simulink model "sm_abbYuMi_trajectory"  (R2025a)
settings: Solver=daessc  StartTime=0.0  StopTime=size(waypointsL,2)*segment_duration  MaxStep=0.5  RelTol=1e-3  AbsTol=1e-3
values from neighbouring files (symbols this model uses):
  cube_l = 0.02    [startup_sm_abbYuMi_trajectory.m]
  segment_duration = 2    [startup_sm_abbYuMi_trajectory.m]
undefined symbols (not defined in the file or in its folder): F1, F2, X, Y, Z
libraries: sm_lib x210, nesl_utility x31, robotcorelib x2
(part 1 of 5)
CloseFcn:
  | try,close(h1_sm_abbYuMi_trajectory),end
  | clear h1_sm_abbYuMi_2_trajectory
  | try,close(h2_sm_abbYuMi_trajectory),end
  | clear h2_sm_abbYuMi_2_trajectory
  | try,close(h3_sm_abbYuMi_trajectory),end
  | clear h3_sm_abbYuMi_2_trajectory
  | try,close(h4_sm_abbYuMi_trajectory),end
  | clear h4_sm_abbYuMi_trajectory
  | 
  | 
  | clear simlog_sm_abbYuMi_trajectory
  | clear logsout_sm_abbYuMi_trajectory
Description:
  | Dual Arm Robot Trajectory Testing
  | Copyright 2021-2025 The MathWorks, Inc.
settings Model: Creator=smiller  LastModifiedBy=smiller
settings SolverCC: AutoScaleAbsTol=off
settings DataIOCC: MaxDataPoints=10000  ReturnWorkspaceOutputs=off  SignalLoggingName=logsout_sm_abbYuMi_trajectory
settings OptimizationCC: ReuseModelBlockBuffer=off
settings DebuggingCC: UnconnectedInputMsg=warning  UnconnectedOutputMsg=warning  UnconnectedLineMsg=warning
settings ModelReferenceCC: EnableRefExpFcnMdlSchedulingChecks=on
settings RTWCC: GPUComputeCapability=3.5  DLArmComputeVersion=19.05
settings SimscapeCC: SimscapeLogType=all  SimscapeLogSimulationStatistics=on  SimscapeLogName=simlog_sm_abbYuMi_trajectory  SimscapeLogDataHistory=10000.0
settings ExplorerConfigSet: InternalSimMechanicsExplorerSettings="<ExplorerConfiguration><canonicalview>default</canonicalview><AnimationSetting><BasePlaybackSpeed>1.0</BasePlaybackSpeed><PlaybackSpeedFactor>1.0</PlaybackSpeedFactor></AnimationSetting><TilePanel><TileInfo><Tiles Columns=\"3\" Count=\"4\" Rows=\"2\"><Column Weight=\"0.6174\"/><Column Weight=\"0.1908\"/><Column Weight=\"0.1918\"/><Row Weight=\"0.4992\"/><Row Weight=\"0.5008\"/><Tile Height=\"2\" Width=\"1\" X=\"0\" Y=\"0\"/><Tile Height=\"1\" Width=\"1\" X=\"1\" Y=\"0\"/><Tile Height=\"1\" Width=\"1\" X=\"2\" Y=\"0\"/><Tile Height=\"1\" Width=\"2\" X=\"1\" Y=\"1\"/></Tiles></TileInfo><SceneInfo><SceneViewer><BGColor><R>1</R><G>1</G><B>1</B></BGColor><Camera><DoPerspective>off</DoPerspective><Position><X>1.10785151491655953</X><Y>0.401938303575801459</Y><Z>0.73930542035196356</Z></Position><Center><X>0.0422085680859981827</X><Y>-0.0186832884618209454</Y><Z>0.276020887594053299</Z></Center><Up><X>-0.346127033108781346</X><Y>-0.144162748431228449</Y><Z>0.927045402834222987</Z></Up><ViewLimDist>1</ViewLimDist><YLim>0.529480286240577747</YLim><XLim>0.750259888990338908</XLim></Camera></SceneViewer><SceneViewer><BGColor><R>1</R><G>1</G><B>1</B></BGColor><Camera><DoPerspective>off</DoPerspective><Position><X>1.28857080950961111</X><Y>0.165761602408297848</Y><Z>0.538044175913367062</Z></Position><Center><X>0.222927862679049932</X><Y>-0.254859989629324657</Y><Z>0.0747596431554567176</Z></Center><Up><X>-0.346127033108781346</X><Y>-0.144162748431228449</Y><Z>0.927045402834222987</Z></Up><ViewLimDist>1</ViewLimDist><YLim>0.0401775125475980072</YLim><XLim>0.0353441275794659157</XLim></Camera></SceneViewer><SceneViewer><BGColor><R>1</R><G>1</G><B>1</B></BGColor><Camera><DoPerspective>off</DoPerspective><Position><X>1.11107526675001367</X><Y>0.699993298566071065</Y><Z>0.461282465118678986</Z></Position><Center><X>0.045432319919452957</X><Y>0.279371706528448394</Y><Z>-0.002002067639231578</Z></Center><Up><X>-0.346127033108781346</X><Y>-0.144162748431228449</Y><Z>0.927045402834222987</Z></Up><ViewLimDist>1</ViewLimDist><YLim>0.0406072638280753281</YLim><XLim>0.0358748383443522681</XLim></Camera></SceneViewer><SceneViewer><BGColor><R>1</R><G>1</G><B>1</B></BGColor><Camera><DoPerspective>off</DoPerspective><Position><X>1.27319716760923374</X><Y>0.344894477488872697</Y><Z>0.410769600840851012</Z></Position><Center><X>0.207554220778672804</X><Y>-0.0757271145487498354</Y><Z>-0.0525149319170593112</Z></Center><Up><X>-0.346127033108781346</X><Y>-0.144162748431228449</Y><Z>0.927045402834222987</Z></Up><ViewLimDist>1</ViewLimDist><YLim>0.0389773841730341117</YLim><XLim>0.0697797364595891534</XLim></Camera></SceneViewer></SceneInfo></TilePanel><MechEditorPanel><Cameras/><GfxPanelCameraMap/><VideoCreator><PlaybackSpeedRatio>1</PlaybackSpeedRatio><FrameRate>30</FrameRate><VideoFormat>MPEG-4</VideoFormat><FrameSize>auto</FrameSize></VideoCreator></MechEditorPanel></ExplorerConfiguration>"

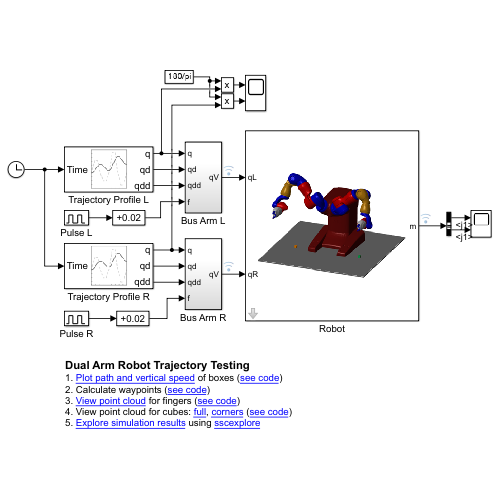
[thumbnail: Simulink's stored preview of the top-level diagram]
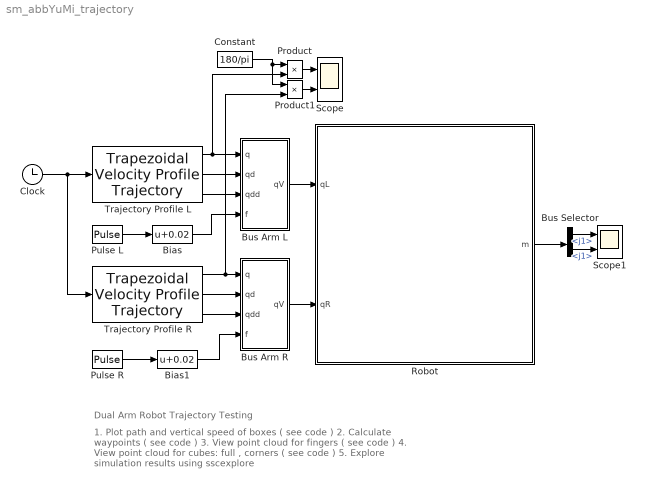
== system sm_abbYuMi_trajectory ==
  note: Dual Arm Robot Trajectory Testing
  note: 1. Plot path and vertical speed of boxes ( see code )
      | 2. Calculate waypoints ( see code )
      | 3. View point cloud for fingers ( see code )
      | 4. View point cloud for cubes: full , corners ( see code )
      | 5. Explore simulation results using sscexplore
  Bias : Bias  Bias=0.02  SaturateOnIntegerOverflow=off
  Bias1 : Bias  Bias=0.02  SaturateOnIntegerOverflow=off
  Bus Selector : BusSelector  OutputSignals=trqL.j1,trqR.j1
  Bus Arm L : Subsystem
  Bus Arm R : Subsystem
  Clock : Clock
  Constant : Constant  Value=180/pi
  Product : Product
  Product1 : Product
  Pulse L : DiscretePulseGenerator  PulseType=Time based  Amplitude=-0.011  Period=100  PulseWidth=4*segment_duration  PhaseDelay=2*segment_duration
  Pulse R : DiscretePulseGenerator  PulseType=Time based  Amplitude=-0.011  Period=100  PulseWidth=4*segment_duration  PhaseDelay=6*segment_duration
  Robot : Subsystem  mask(Dual Arm Robot with Contact Forces){k_gripBox=1e3, k_boxBox=1e3, k_boxFloor=1e3, d_gripBox=1e2, d_boxBox=1e2, d_boxFloor=1e2, t_gripBox=1e-3, t_boxBox=1e-3, t_boxFloor=1e-3, mu_s_gripBox=0.7, mu_s_boxBox=0.5, mu_s_boxFloor=0.5, mu_d_gripBox=0.5, mu_d_boxBox=0.3, mu_d_boxFloor=0.3, mu_v_gripBox=1e-3, mu_v_boxBox=1e-3, mu_v_boxFloor=1e-3}
      mask help: Models a dual-arm robot. Parameter values define the contact and friction forces between the gripper, boxes, and floor.
      mask DialogControl Control2_copy_copy_copy_copy_copy_copy_copy Prompt: Gripper-Box
      mask DialogControl Control2_copy_copy_copy_copy_copy_copy_copy_copy Prompt: Box-Box
      mask DialogControl Control2_copy_copy_copy_copy_copy_copy_copy_copy_copy Prompt: Box-Floor
      mask DialogControl Control2_copy_copy_copy_copy_copy_copy Prompt: Damping (N/(m/s))
      mask DialogControl Control2_copy Prompt: Damping (N/(m/s))
      mask DialogControl Control2_copy_copy Prompt: Transition Width (m)
      mask DialogControl Control2_copy_copy_copy Prompt: Static Friction (0-1)
      mask DialogControl Control2_copy_copy_copy_copy Prompt: Dynamic Friction (0-1)
      mask DialogControl Control2_copy_copy_copy_copy_copy Prompt: Critical Velocity (m/s)
      mask Display: image('sm_abbYuMi_trajectory_robot.png');
  Scope : Scope  NumInputPorts=2
      settings: ActiveDisplayYMinimum=-224.28794  ActiveDisplayYMaximum=180.85767
  Scope1 : Scope  NumInputPorts=2
      settings: ActiveDisplayYMinimum=-24.11191  ActiveDisplayYMaximum=24.30925
  Trajectory Profile L : robotcorelib/Trapezoidal Velocity Profile Trajectory  WaypointSource=Internal  Waypoints=waypointsL  NumParams=1  Parameter1=End Time  Parameter2=End Time  ParameterSource=Internal  PeakVelocity=[ 2; 2 ]  Acceleration=[ 1; 2 ]  EndTime=segment_duration  AccelTime=[ 1; 2 ]  SimulateUsing=Code generation
  Trajectory Profile R : robotcorelib/Trapezoidal Velocity Profile Trajectory  WaypointSource=Internal  Waypoints=waypointsR  NumParams=1  Parameter1=End Time  Parameter2=End Time  ParameterSource=Internal  PeakVelocity=[ 2; 2 ]  Acceleration=[ 1; 2 ]  EndTime=segment_duration  AccelTime=[ 1; 2 ]  SimulateUsing=Code generation
  wires:
  Clock/1 -> Trajectory Profile R/1, Trajectory Profile L/1
  Trajectory Profile L/1 -> Product/2, Bus Arm L/1(q)
  Trajectory Profile L/2 -> Bus Arm L/2(qd)
  Trajectory Profile L/3 -> Bus Arm L/3(qdd)
  Product/1 -> Scope/1
  Pulse L/1 -> Bias/1
  Trajectory Profile R/3 -> Bus Arm R/3(qdd)
  Trajectory Profile R/2 -> Bus Arm R/2(qd)
  Trajectory Profile R/1 -> Product1/2, Bus Arm R/1(q)
  Product1/1 -> Scope/2
  Pulse R/1 -> Bias1/1
  Bus Arm L/1(qV) -> Robot/1(qL)
  Bus Arm R/1(qV) -> Robot/2(qR)
  Constant/1 -> Product1/1, Product/1
  Bias1/1 -> Bus Arm R/4(f)
  Bias/1 -> Bus Arm L/4(f)
  Robot/1(m) -> Bus Selector/1
  Bus Selector/1 -> Scope1/1  "<j1>"
  Bus Selector/2 -> Scope1/2  "<j1>"

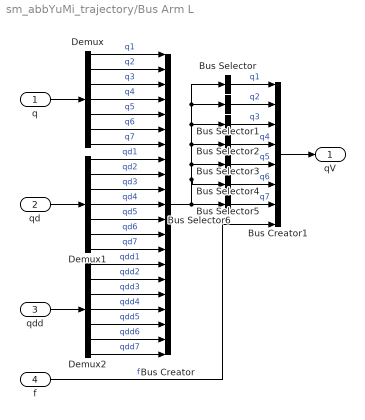
== system sm_abbYuMi_trajectory/Bus Arm L ==
  q : Inport
  qd : Inport  Port=2
  qdd : Inport  Port=3
  f : Inport  Port=4
  Bus Creator : BusCreator  Inputs=21
  Bus Creator1 : BusCreator  Inputs=8
  Bus Selector : BusSelector  OutputSignals=q1,qd1,qdd1  OutputAsBus=on
  Bus Selector1 : BusSelector  OutputSignals=q2,qd2,qdd2  OutputAsBus=on
  Bus Selector2 : BusSelector  OutputSignals=q3,qd3,qdd3  OutputAsBus=on
  Bus Selector3 : BusSelector  OutputSignals=q4,qd4,qdd4  OutputAsBus=on
  Bus Selector4 : BusSelector  OutputSignals=q5,qd5,qdd5  OutputAsBus=on
  Bus Selector5 : BusSelector  OutputSignals=q6,qd6,qdd6  OutputAsBus=on
  Bus Selector6 : BusSelector  OutputSignals=q7,qd7,qdd7  OutputAsBus=on
  Demux : Demux  Outputs=7
  Demux1 : Demux  Outputs=7
  Demux2 : Demux  Outputs=7
  qV : Outport
  wires:
  f/1 -> Bus Creator1/8  "f"
  q/1 -> Demux/1
  qd/1 -> Demux1/1
  qdd/1 -> Demux2/1
  Demux/1 -> Bus Creator/1  "q1"
  Demux/2 -> Bus Creator/2  "q2"
  Demux/3 -> Bus Creator/3  "q3"
  Demux/4 -> Bus Creator/4  "q4"
  Demux/5 -> Bus Creator/5  "q5"
  Demux/6 -> Bus Creator/6  "q6"
  Demux/7 -> Bus Creator/7  "q7"
  Demux1/1 -> Bus Creator/8  "qd1"
  Demux1/2 -> Bus Creator/9  "qd2"
  Demux1/3 -> Bus Creator/10  "qd3"
  Demux1/4 -> Bus Creator/11  "qd4"
  Demux1/5 -> Bus Creator/12  "qd5"
  Demux1/6 -> Bus Creator/13  "qd6"
  Demux1/7 -> Bus Creator/14  "qd7"
  Demux2/1 -> Bus Creator/15  "qdd1"
  Demux2/2 -> Bus Creator/16  "qdd2"
  Demux2/3 -> Bus Creator/17  "qdd3"
  Demux2/4 -> Bus Creator/18  "qdd4"
  Demux2/5 -> Bus Creator/19  "qdd5"
  Demux2/6 -> Bus Creator/20  "qdd6"
  Demux2/7 -> Bus Creator/21  "qdd7"
  Bus Creator/1 -> Bus Selector5/1, Bus Selector4/1, Bus Selector3/1, Bus Selector2/1, Bus Selector/1, Bus Selector1/1, Bus Selector6/1
  Bus Selector/1 -> Bus Creator1/1  "q1"
  Bus Selector1/1 -> Bus Creator1/2  "q2"
  Bus Selector2/1 -> Bus Creator1/3  "q3"
  Bus Selector3/1 -> Bus Creator1/4  "q4"
  Bus Selector4/1 -> Bus Creator1/5  "q5"
  Bus Selector5/1 -> Bus Creator1/6  "q6"
  Bus Selector6/1 -> Bus Creator1/7  "q7"
  Bus Creator1/1 -> qV/1

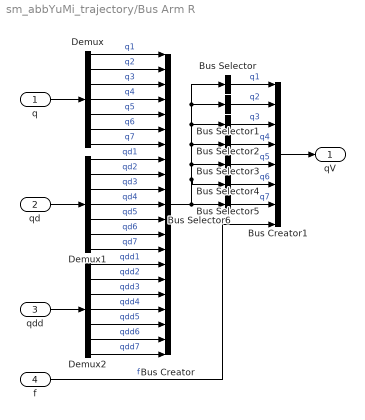
== system sm_abbYuMi_trajectory/Bus Arm R ==
  q : Inport
  qd : Inport  Port=2
  qdd : Inport  Port=3
  f : Inport  Port=4
  Bus Creator : BusCreator  Inputs=21
  Bus Creator1 : BusCreator  Inputs=8
  Bus Selector : BusSelector  OutputSignals=q1,qd1,qdd1  OutputAsBus=on
  Bus Selector1 : BusSelector  OutputSignals=q2,qd2,qdd2  OutputAsBus=on
  Bus Selector2 : BusSelector  OutputSignals=q3,qd3,qdd3  OutputAsBus=on
  Bus Selector3 : BusSelector  OutputSignals=q4,qd4,qdd4  OutputAsBus=on
  Bus Selector4 : BusSelector  OutputSignals=q5,qd5,qdd5  OutputAsBus=on
  Bus Selector5 : BusSelector  OutputSignals=q6,qd6,qdd6  OutputAsBus=on
  Bus Selector6 : BusSelector  OutputSignals=q7,qd7,qdd7  OutputAsBus=on
  Demux : Demux  Outputs=7
  Demux1 : Demux  Outputs=7
  Demux2 : Demux  Outputs=7
  qV : Outport
  wires:
  Bus Creator1/1 -> qV/1
  Bus Selector6/1 -> Bus Creator1/7  "q7"
  Bus Selector5/1 -> Bus Creator1/6  "q6"
  Bus Selector4/1 -> Bus Creator1/5  "q5"
  Bus Selector3/1 -> Bus Creator1/4  "q4"
  Bus Selector2/1 -> Bus Creator1/3  "q3"
  Bus Selector1/1 -> Bus Creator1/2  "q2"
  Bus Selector/1 -> Bus Creator1/1  "q1"
  Bus Creator/1 -> Bus Selector6/1, Bus Selector1/1, Bus Selector/1, Bus Selector2/1, Bus Selector3/1, Bus Selector4/1, Bus Selector5/1
  Demux2/7 -> Bus Creator/21  "qdd7"
  Demux2/6 -> Bus Creator/20  "qdd6"
  Demux2/5 -> Bus Creator/19  "qdd5"
  Demux2/4 -> Bus Creator/18  "qdd4"
  Demux2/3 -> Bus Creator/17  "qdd3"
  Demux2/2 -> Bus Creator/16  "qdd2"
  Demux2/1 -> Bus Creator/15  "qdd1"
  Demux1/7 -> Bus Creator/14  "qd7"
  Demux1/6 -> Bus Creator/13  "qd6"
  Demux1/5 -> Bus Creator/12  "qd5"
  Demux1/4 -> Bus Creator/11  "qd4"
  Demux1/3 -> Bus Creator/10  "qd3"
  Demux1/2 -> Bus Creator/9  "qd2"
  Demux1/1 -> Bus Creator/8  "qd1"
  Demux/7 -> Bus Creator/7  "q7"
  Demux/6 -> Bus Creator/6  "q6"
  Demux/5 -> Bus Creator/5  "q5"
  Demux/4 -> Bus Creator/4  "q4"
  Demux/3 -> Bus Creator/3  "q3"
  Demux/2 -> Bus Creator/2  "q2"
  Demux/1 -> Bus Creator/1  "q1"
  qdd/1 -> Demux2/1
  qd/1 -> Demux1/1
  q/1 -> Demux/1
  f/1 -> Bus Creator1/8  "f"

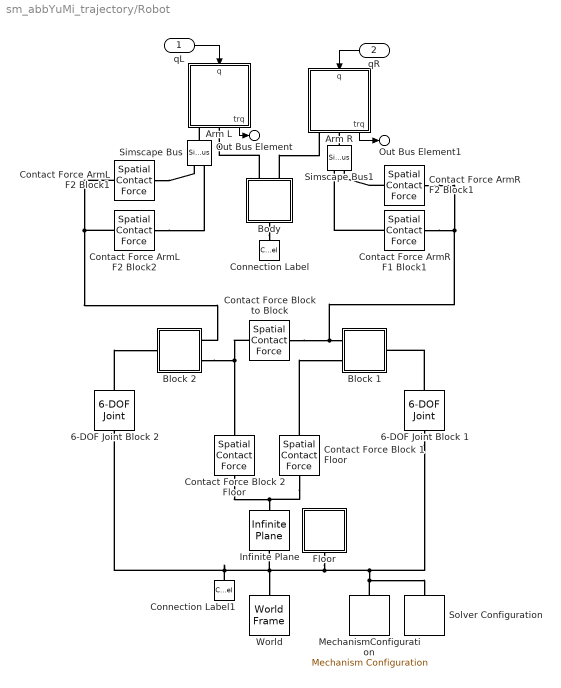
== system sm_abbYuMi_trajectory/Robot ==
  qL : Inport
  qR : Inport  Port=2
  " Contact Force Block to Block" : sm_lib/Forces and Torques/Spatial Contact Force  SenseSeparationDistance=off  NormalForceType=SmoothSpringDamper  NormalStiffness=k_boxBox  NormalStiffnessUnits=N/m  NormalDamping=d_boxBox  NormalDampingUnits=N/(m/s)  NormalTransitionRegionWidth=t_boxBox  NormalTransitionRegionWidthUnits=m  FrictionType=SmoothStickSlip  CoefficientOfStaticFriction=mu_s_boxBox  CoefficientOfDynamicFriction=mu_d_boxBox  FrictionalCriticalVelocity=mu_v_boxBox  FrictionalCriticalVelocityUnits=m/s  SenseContactSignal=off  SensePenetrationDepth=off  SenseNormalVelocity=off  SenseTangentialVelocity=off  SensingForceTorqueDirection=BaseOnFollower  SensingForceTorqueResolutionFrame=ContactFrame  SenseNormalForce=off  SenseNormalForceMagnitude=off  SenseNormalTorque=off  SenseFrictionalForce=off  SenseFrictionalForceMagnitude=off  SenseFrictionalTorque=off  SenseTotalForce=off  SenseTotalTorque=off  SenseContactBaseRotation=off  SenseContactBaseTranslation=off  SenseContactFollowerRotation=off  SenseContactFollowerTranslation=off  ZeroCrossDetectContactStartAndEnd=off
  6-DOF Joint Block 1 : sm_lib/Joints/6-DOF Joint  JointMode=Normal  CompositeWrenchDir=FollowerOnBase  CompositeWrenchFrame=BaseFrame  SenseConstraintForce=off  SenseConstraintTorque=off  SenseTotalForce=off  SenseTotalTorque=off  PxPositionTargetSpecify=on  PxPositionTargetPriority=High  PxPositionTargetValue=0.1  PxPositionTargetValueUnits=m  PxVelocityTargetSpecify=off  PxVelocityTargetPriority=High  PxVelocityTargetValue=0  PxVelocityTargetValueUnits=m/s  PxEquilibriumPosition=0  PxEquilibriumPositionUnits=m  PxSpringStiffness=0  PxSpringStiffnessUnits=N/m  PxDampingCoefficient=0  PxDampingCoefficientUnits=N/(m/s)  PxLowerLimitSpecify=off  PxLowerLimitBound=-1  PxLowerLimitBoundUnits=m  PxLowerLimitStiffness=1e6  PxLowerLimitStiffnessUnits=N/m  PxLowerLimitDamping=1e3  PxLowerLimitDampingUnits=N/(m/s)  PxLowerLimitTransitionRegionWidth=1e-4  PxLowerLimitTransitionRegionWidthUnits=m  PxUpperLimitSpecify=off  PxUpperLimitBound=1  PxUpperLimitBoundUnits=m  PxUpperLimitStiffness=1e6  PxUpperLimitStiffnessUnits=N/m  PxUpperLimitDamping=1e3  PxUpperLimitDampingUnits=N/(m/s)  PxUpperLimitTransitionRegionWidth=1e-4  PxUpperLimitTransitionRegionWidthUnits=m  PxTorqueActuationMode=NoTorque  PxMotionActuationMode=ComputedMotion  PxSensePosition=off  PxSenseVelocity=off  PxSenseAcceleration=off  PxSenseTorqueForce=off  PxSenseLowerLimitTorqueForce=off  PxSenseUpperLimitTorqueForce=off  PyPositionTargetSpecify=on  PyPositionTargetPriority=High  PyPositionTargetValue=-0.3  PyPositionTargetValueUnits=m  PyVelocityTargetSpecify=off  PyVelocityTargetPriority=High  PyVelocityTargetValue=0  PyVelocityTargetValueUnits=m/s  PyEquilibriumPosition=0  PyEquilibriumPositionUnits=m  PySpringStiffness=0  PySpringStiffnessUnits=N/m  PyDampingCoefficient=0  PyDampingCoefficientUnits=N/(m/s)  PyLowerLimitSpecify=off  PyLowerLimitBound=-1  PyLowerLimitBoundUnits=m  PyLowerLimitStiffness=1e6  PyLowerLimitStiffnessUnits=N/m  PyLowerLimitDamping=1e3  PyLowerLimitDampingUnits=N/(m/s)  PyLowerLimitTransitionRegionWidth=1e-4  PyLowerLimitTransitionRegionWidthUnits=m  PyUpperLimitSpecify=off  PyUpperLimitBound=1  PyUpperLimitBoundUnits=m  PyUpperLimitStiffness=1e6  PyUpperLimitStiffnessUnits=N/m  PyUpperLimitDamping=1e3  PyUpperLimitDampingUnits=N/(m/s)  PyUpperLimitTransitionRegionWidth=1e-4  PyUpperLimitTransitionRegionWidthUnits=m  PyTorqueActuationMode=NoTorque  PyMotionActuationMode=ComputedMotion  PySensePosition=off  PySenseVelocity=off  PySenseAcceleration=off  PySenseTorqueForce=off  PySenseLowerLimitTorqueForce=off  PySenseUpperLimitTorqueForce=off  PzPositionTargetSpecify=on  PzPositionTargetPriority=High  PzPositionTargetValue=0.011  PzPositionTargetValueUnits=m  PzVelocityTargetSpecify=off  PzVelocityTargetPriority=High  PzVelocityTargetValue=0  PzVelocityTargetValueUnits=m/s  PzEquilibriumPosition=0  PzEquilibriumPositionUnits=m  PzSpringStiffness=0  PzSpringStiffnessUnits=N/m  PzDampingCoefficient=0  PzDampingCoefficientUnits=N/(m/s)  PzLowerLimitSpecify=off  PzLowerLimitBound=0  PzLowerLimitBoundUnits=m  PzLowerLimitStiffness=1e6  PzLowerLimitStiffnessUnits=N/m  PzLowerLimitDamping=1e3  PzLowerLimitDampingUnits=N/(m/s)  PzLowerLimitTransitionRegionWidth=1e-4  PzLowerLimitTransitionRegionWidthUnits=m  PzUpperLimitSpecify=off  PzUpperLimitBound=1  PzUpperLimitBoundUnits=m  PzUpperLimitStiffness=1e6  PzUpperLimitStiffnessUnits=N/m  PzUpperLimitDamping=1e3  PzUpperLimitDampingUnits=N/(m/s)  PzUpperLimitTransitionRegionWidth=1e-4  PzUpperLimitTransitionRegionWidthUnits=m  PzTorqueActuationMode=NoTorque  PzMotionActuationMode=ComputedMotion  PzSensePosition=off  PzSenseVelocity=off  PzSenseAcceleration=off  PzSenseTorqueForce=off  PzSenseLowerLimitTorqueForce=off  PzSenseUpperLimitTorqueForce=off  SphPositionTargetSpecify=off  SphPositionTargetPriority=High  SphPositionTargetRotationMethod=None  SphPositionTargetFollAlignAxisA=+X  SphPositionTargetBaseAlignAxisA=+Y  SphPositionTargetFollAlignAxisB=+Y  SphPositionTargetBaseAlignAxisB=+Z  SphPositionTargetRotationStandardAxis=+Z  SphPositionTargetRotationAngle=0.0  SphPositionTargetRotationAngleUnits=deg  SphPositionTargetRotationArbitraryAxis=[0 0 1]  SphPositionTargetRotationSequenceAxes=FollowerAxes  SphPositionTargetRotationSequence=XYX  SphPositionTargetRotationSequenceAngles=[0 0 0]  SphPositionTargetRotationSequenceAnglesUnits=deg  SphPositionTargetRotationMatrix=[1 0 0; 0 1 0; 0 0 1]  SphPositionTargetQuaternion=[1 0 0 0]  SphVelocityTargetSpecify=off  SphVelocityTargetPriority=High  SphVelocityTargetValue=[0 0 0]  SphVelocityTargetValueUnits=deg/s  SphVelocityTargetInFollowerFrame=on  SphEqPosRotationMethod=None  SphEqPosFollAlignAxisA=+X  SphEqPosBaseAlignAxisA=+Y  SphEqPosFollAlignAxisB=+Y  SphEqPosBaseAlignAxisB=+Z  SphEqPosRotationStandardAxis=+Z  SphEqPosRotationAngle=0.0  SphEqPosRotationAngleUnits=deg  SphEqPosRotationArbitraryAxis=[0 0 1]  SphEqPosRotationSequenceAxes=FollowerAxes  SphEqPosRotationSequence=XYX  SphEqPosRotationSequenceAngles=[0 0 0]  SphEqPosRotationSequenceAnglesUnits=deg  SphEqPosRotationMatrix=[1 0 0; 0 1 0; 0 0 1]  SphEqPosQuaternion=[1 0 0 0]  SphSpringStiffness=0  SphSpringStiffnessUnits=N*m/deg  SphDampingCoefficient=0  SphDampingCoefficientUnits=N*m/(deg/s)  SphLowerLimitSpecify=off  SphLowerLimitBound=15  SphLowerLimitBoundUnits=deg  SphLowerLimitStiffness=1e4  SphLowerLimitStiffnessUnits=N*m/deg  SphLowerLimitDamping=10  SphLowerLimitDampingUnits=N*m/(deg/s)  SphLowerLimitTransitionRegionWidth=0.1  SphLowerLimitTransitionRegionWidthUnits=deg  SphUpperLimitSpecify=off  SphUpperLimitBound=45  SphUpperLimitBoundUnits=deg  SphUpperLimitStiffness=1e4  SphUpperLimitStiffnessUnits=N*m/deg  SphUpperLimitDamping=10  SphUpperLimitDampingUnits=N*m/(deg/s)  SphUpperLimitTransitionRegionWidth=0.1  SphUpperLimitTransitionRegionWidthUnits=deg  SphTorqueActuationMode=NoTorque  SphActuateTorqueX=off  SphActuateTorqueY=off  SphActuateTorqueZ=off  SphActuateTorque=off  SphActuationFrame=BaseFrame  SphSensePosition=off  SphSenseVelocityX=off  SphSenseVelocityY=off  SphSenseVelocityZ=off  SphSenseVelocity=off  SphSenseAccelerationX=off  SphSenseAccelerationY=off  SphSenseAccelerationZ=off  SphSenseAcceleration=off  SphSenseLowerLimitTorqueMag=off  SphSenseUpperLimitTorqueMag=off  SphSensingFrame=BaseFrame
  6-DOF Joint Block 2 : sm_lib/Joints/6-DOF Joint  JointMode=Normal  CompositeWrenchDir=FollowerOnBase  CompositeWrenchFrame=BaseFrame  SenseConstraintForce=off  SenseConstraintTorque=off  SenseTotalForce=off  SenseTotalTorque=off  PxPositionTargetSpecify=on  PxPositionTargetPriority=High  PxPositionTargetValue=0.1  PxPositionTargetValueUnits=m  PxVelocityTargetSpecify=off  PxVelocityTargetPriority=High  PxVelocityTargetValue=0  PxVelocityTargetValueUnits=m/s  PxEquilibriumPosition=0  PxEquilibriumPositionUnits=m  PxSpringStiffness=0  PxSpringStiffnessUnits=N/m  PxDampingCoefficient=0  PxDampingCoefficientUnits=N/(m/s)  PxLowerLimitSpecify=off  PxLowerLimitBound=-1  PxLowerLimitBoundUnits=m  PxLowerLimitStiffness=1e6  PxLowerLimitStiffnessUnits=N/m  PxLowerLimitDamping=1e3  PxLowerLimitDampingUnits=N/(m/s)  PxLowerLimitTransitionRegionWidth=1e-4  PxLowerLimitTransitionRegionWidthUnits=m  PxUpperLimitSpecify=off  PxUpperLimitBound=1  PxUpperLimitBoundUnits=m  PxUpperLimitStiffness=1e6  PxUpperLimitStiffnessUnits=N/m  PxUpperLimitDamping=1e3  PxUpperLimitDampingUnits=N/(m/s)  PxUpperLimitTransitionRegionWidth=1e-4  PxUpperLimitTransitionRegionWidthUnits=m  PxTorqueActuationMode=NoTorque  PxMotionActuationMode=ComputedMotion  PxSensePosition=off  PxSenseVelocity=off  PxSenseAcceleration=off  PxSenseTorqueForce=off  PxSenseLowerLimitTorqueForce=off  PxSenseUpperLimitTorqueForce=off  PyPositionTargetSpecify=on  PyPositionTargetPriority=High  PyPositionTargetValue=0.3  PyPositionTargetValueUnits=m  PyVelocityTargetSpecify=off  PyVelocityTargetPriority=High  PyVelocityTargetValue=0  PyVelocityTargetValueUnits=m/s  PyEquilibriumPosition=0  PyEquilibriumPositionUnits=m  PySpringStiffness=0  PySpringStiffnessUnits=N/m  PyDampingCoefficient=0  PyDampingCoefficientUnits=N/(m/s)  PyLowerLimitSpecify=off  PyLowerLimitBound=-1  PyLowerLimitBoundUnits=m  PyLowerLimitStiffness=1e6  PyLowerLimitStiffnessUnits=N/m  PyLowerLimitDamping=1e3  PyLowerLimitDampingUnits=N/(m/s)  PyLowerLimitTransitionRegionWidth=1e-4  PyLowerLimitTransitionRegionWidthUnits=m  PyUpperLimitSpecify=off  PyUpperLimitBound=1  PyUpperLimitBoundUnits=m  PyUpperLimitStiffness=1e6  PyUpperLimitStiffnessUnits=N/m  PyUpperLimitDamping=1e3  PyUpperLimitDampingUnits=N/(m/s)  PyUpperLimitTransitionRegionWidth=1e-4  PyUpperLimitTransitionRegionWidthUnits=m  PyTorqueActuationMode=NoTorque  PyMotionActuationMode=ComputedMotion  PySensePosition=off  PySenseVelocity=off  PySenseAcceleration=off  PySenseTorqueForce=off  PySenseLowerLimitTorqueForce=off  PySenseUpperLimitTorqueForce=off  PzPositionTargetSpecify=on  PzPositionTargetPriority=High  PzPositionTargetValue=0.011  PzPositionTargetValueUnits=m  PzVelocityTargetSpecify=off  PzVelocityTargetPriority=High  PzVelocityTargetValue=0  PzVelocityTargetValueUnits=m/s  PzEquilibriumPosition=0  PzEquilibriumPositionUnits=m  PzSpringStiffness=0  PzSpringStiffnessUnits=N/m  PzDampingCoefficient=0  PzDampingCoefficientUnits=N/(m/s)  PzLowerLimitSpecify=off  PzLowerLimitBound=0  PzLowerLimitBoundUnits=m  PzLowerLimitStiffness=1e6  PzLowerLimitStiffnessUnits=N/m  PzLowerLimitDamping=1e3  PzLowerLimitDampingUnits=N/(m/s)  PzLowerLimitTransitionRegionWidth=1e-4  PzLowerLimitTransitionRegionWidthUnits=m  PzUpperLimitSpecify=off  PzUpperLimitBound=1  PzUpperLimitBoundUnits=m  PzUpperLimitStiffness=1e6  PzUpperLimitStiffnessUnits=N/m  PzUpperLimitDamping=1e3  PzUpperLimitDampingUnits=N/(m/s)  PzUpperLimitTransitionRegionWidth=1e-4  PzUpperLimitTransitionRegionWidthUnits=m  PzTorqueActuationMode=NoTorque  PzMotionActuationMode=ComputedMotion  PzSensePosition=off  PzSenseVelocity=off  PzSenseAcceleration=off  PzSenseTorqueForce=off  PzSenseLowerLimitTorqueForce=off  PzSenseUpperLimitTorqueForce=off  SphPositionTargetSpecify=off  SphPositionTargetPriority=High  SphPositionTargetRotationMethod=None  SphPositionTargetFollAlignAxisA=+X  SphPositionTargetBaseAlignAxisA=+Y  SphPositionTargetFollAlignAxisB=+Y  SphPositionTargetBaseAlignAxisB=+Z  SphPositionTargetRotationStandardAxis=+Z  SphPositionTargetRotationAngle=0.0  SphPositionTargetRotationAngleUnits=deg  SphPositionTargetRotationArbitraryAxis=[0 0 1]  SphPositionTargetRotationSequenceAxes=FollowerAxes  SphPositionTargetRotationSequence=XYX  SphPositionTargetRotationSequenceAngles=[0 0 0]  SphPositionTargetRotationSequenceAnglesUnits=deg  SphPositionTargetRotationMatrix=[1 0 0; 0 1 0; 0 0 1]  SphPositionTargetQuaternion=[1 0 0 0]  SphVelocityTargetSpecify=off  SphVelocityTargetPriority=High  SphVelocityTargetValue=[0 0 0]  SphVelocityTargetValueUnits=deg/s  SphVelocityTargetInFollowerFrame=on  SphEqPosRotationMethod=None  SphEqPosFollAlignAxisA=+X  SphEqPosBaseAlignAxisA=+Y  SphEqPosFollAlignAxisB=+Y  SphEqPosBaseAlignAxisB=+Z  SphEqPosRotationStandardAxis=+Z  SphEqPosRotationAngle=0.0  SphEqPosRotationAngleUnits=deg  SphEqPosRotationArbitraryAxis=[0 0 1]  SphEqPosRotationSequenceAxes=FollowerAxes  SphEqPosRotationSequence=XYX  SphEqPosRotationSequenceAngles=[0 0 0]  SphEqPosRotationSequenceAnglesUnits=deg  SphEqPosRotationMatrix=[1 0 0; 0 1 0; 0 0 1]  SphEqPosQuaternion=[1 0 0 0]  SphSpringStiffness=0  SphSpringStiffnessUnits=N*m/deg  SphDampingCoefficient=0  SphDampingCoefficientUnits=N*m/(deg/s)  SphLowerLimitSpecify=off  SphLowerLimitBound=15  SphLowerLimitBoundUnits=deg  SphLowerLimitStiffness=1e4  SphLowerLimitStiffnessUnits=N*m/deg  SphLowerLimitDamping=10  SphLowerLimitDampingUnits=N*m/(deg/s)  SphLowerLimitTransitionRegionWidth=0.1  SphLowerLimitTransitionRegionWidthUnits=deg  SphUpperLimitSpecify=off  SphUpperLimitBound=45  SphUpperLimitBoundUnits=deg  SphUpperLimitStiffness=1e4  SphUpperLimitStiffnessUnits=N*m/deg  SphUpperLimitDamping=10  SphUpperLimitDampingUnits=N*m/(deg/s)  SphUpperLimitTransitionRegionWidth=0.1  SphUpperLimitTransitionRegionWidthUnits=deg  SphTorqueActuationMode=NoTorque  SphActuateTorqueX=off  SphActuateTorqueY=off  SphActuateTorqueZ=off  SphActuateTorque=off  SphActuationFrame=BaseFrame  SphSensePosition=off  SphSenseVelocityX=off  SphSenseVelocityY=off  SphSenseVelocityZ=off  SphSenseVelocity=off  SphSenseAccelerationX=off  SphSenseAccelerationY=off  SphSenseAccelerationZ=off  SphSenseAcceleration=off  SphSenseLowerLimitTorqueMag=off  SphSenseUpperLimitTorqueMag=off  SphSensingFrame=BaseFrame
  Arm L : Subsystem
  Arm R : Subsystem
  Block 1 : Subsystem
  Block 2 : Subsystem
  Body : Subsystem
  Connection Label : ConnectionLabel  Label=W
  Connection Label1 : ConnectionLabel  Label=W
  Contact Force Block 1 Floor : sm_lib/Forces and Torques/Spatial Contact Force  SenseSeparationDistance=off  NormalForceType=SmoothSpringDamper  NormalStiffness=k_boxFloor  NormalStiffnessUnits=N/m  NormalDamping=d_boxFloor  NormalDampingUnits=N/(m/s)  NormalTransitionRegionWidth=t_boxFloor  NormalTransitionRegionWidthUnits=m  FrictionType=SmoothStickSlip  CoefficientOfStaticFriction=mu_s_boxFloor  CoefficientOfDynamicFriction=mu_d_boxFloor  FrictionalCriticalVelocity=mu_v_boxFloor  FrictionalCriticalVelocityUnits=m/s  SenseContactSignal=off  SensePenetrationDepth=off  SenseNormalVelocity=off  SenseTangentialVelocity=off  SensingForceTorqueDirection=BaseOnFollower  SensingForceTorqueResolutionFrame=ContactFrame  SenseNormalForce=off  SenseNormalForceMagnitude=off  SenseNormalTorque=off  SenseFrictionalForce=off  SenseFrictionalForceMagnitude=off  SenseFrictionalTorque=off  SenseTotalForce=off  SenseTotalTorque=off  SenseContactBaseRotation=off  SenseContactBaseTranslation=off  SenseContactFollowerRotation=off  SenseContactFollowerTranslation=off  ZeroCrossDetectContactStartAndEnd=off
  Contact Force Block 2 Floor : sm_lib/Forces and Torques/Spatial Contact Force  SenseSeparationDistance=off  NormalForceType=SmoothSpringDamper  NormalStiffness=k_boxFloor  NormalStiffnessUnits=N/m  NormalDamping=d_boxFloor  NormalDampingUnits=N/(m/s)  NormalTransitionRegionWidth=t_boxFloor  NormalTransitionRegionWidthUnits=m  FrictionType=SmoothStickSlip  CoefficientOfStaticFriction=mu_s_boxFloor  CoefficientOfDynamicFriction=mu_d_boxFloor  FrictionalCriticalVelocity=mu_v_boxFloor  FrictionalCriticalVelocityUnits=m/s  SenseContactSignal=off  SensePenetrationDepth=off  SenseNormalVelocity=off  SenseTangentialVelocity=off  SensingForceTorqueDirection=BaseOnFollower  SensingForceTorqueResolutionFrame=ContactFrame  SenseNormalForce=off  SenseNormalForceMagnitude=off  SenseNormalTorque=off  SenseFrictionalForce=off  SenseFrictionalForceMagnitude=off  SenseFrictionalTorque=off  SenseTotalForce=off  SenseTotalTorque=off  SenseContactBaseRotation=off  SenseContactBaseTranslation=off  SenseContactFollowerRotation=off  SenseContactFollowerTranslation=off  ZeroCrossDetectContactStartAndEnd=off
  Contact Force ArmL F2 Block1 : sm_lib/Forces and Torques/Spatial Contact Force  SenseSeparationDistance=off  NormalForceType=SmoothSpringDamper  NormalStiffness=k_gripBox  NormalStiffnessUnits=N/m  NormalDamping=d_gripBox  NormalDampingUnits=N/(m/s)  NormalTransitionRegionWidth=t_gripBox  NormalTransitionRegionWidthUnits=m  FrictionType=SmoothStickSlip  CoefficientOfStaticFriction=mu_s_gripBox  CoefficientOfDynamicFriction=mu_d_gripBox  FrictionalCriticalVelocity=mu_v_gripBox  FrictionalCriticalVelocityUnits=m/s  SenseContactSignal=off  SensePenetrationDepth=off  SenseNormalVelocity=off  SenseTangentialVelocity=off  SensingForceTorqueDirection=BaseOnFollower  SensingForceTorqueResolutionFrame=ContactFrame  SenseNormalForce=off  SenseNormalForceMagnitude=off  SenseNormalTorque=off  SenseFrictionalForce=off  SenseFrictionalForceMagnitude=off  SenseFrictionalTorque=off  SenseTotalForce=off  SenseTotalTorque=off  SenseContactBaseRotation=off  SenseContactBaseTranslation=off  SenseContactFollowerRotation=off  SenseContactFollowerTranslation=off  ZeroCrossDetectContactStartAndEnd=off
  Contact Force ArmL F2 Block2 : sm_lib/Forces and Torques/Spatial Contact Force  SenseSeparationDistance=off  NormalForceType=SmoothSpringDamper  NormalStiffness=k_gripBox  NormalStiffnessUnits=N/m  NormalDamping=d_gripBox  NormalDampingUnits=N/(m/s)  NormalTransitionRegionWidth=t_gripBox  NormalTransitionRegionWidthUnits=m  FrictionType=SmoothStickSlip  CoefficientOfStaticFriction=mu_s_gripBox  CoefficientOfDynamicFriction=mu_d_gripBox  FrictionalCriticalVelocity=mu_v_gripBox  FrictionalCriticalVelocityUnits=m/s  SenseContactSignal=off  SensePenetrationDepth=off  SenseNormalVelocity=off  SenseTangentialVelocity=off  SensingForceTorqueDirection=BaseOnFollower  SensingForceTorqueResolutionFrame=ContactFrame  SenseNormalForce=off  SenseNormalForceMagnitude=off  SenseNormalTorque=off  SenseFrictionalForce=off  SenseFrictionalForceMagnitude=off  SenseFrictionalTorque=off  SenseTotalForce=off  SenseTotalTorque=off  SenseContactBaseRotation=off  SenseContactBaseTranslation=off  SenseContactFollowerRotation=off  SenseContactFollowerTranslation=off  ZeroCrossDetectContactStartAndEnd=off
  Contact Force ArmR F1 Block1 : sm_lib/Forces and Torques/Spatial Contact Force  SenseSeparationDistance=off  NormalForceType=SmoothSpringDamper  NormalStiffness=k_gripBox  NormalStiffnessUnits=N/m  NormalDamping=d_gripBox  NormalDampingUnits=N/(m/s)  NormalTransitionRegionWidth=t_gripBox  NormalTransitionRegionWidthUnits=m  FrictionType=SmoothStickSlip  CoefficientOfStaticFriction=mu_s_gripBox  CoefficientOfDynamicFriction=mu_d_gripBox  FrictionalCriticalVelocity=mu_v_gripBox  FrictionalCriticalVelocityUnits=m/s  SenseContactSignal=off  SensePenetrationDepth=off  SenseNormalVelocity=off  SenseTangentialVelocity=off  SensingForceTorqueDirection=BaseOnFollower  SensingForceTorqueResolutionFrame=ContactFrame  SenseNormalForce=off  SenseNormalForceMagnitude=off  SenseNormalTorque=off  SenseFrictionalForce=off  SenseFrictionalForceMagnitude=off  SenseFrictionalTorque=off  SenseTotalForce=off  SenseTotalTorque=off  SenseContactBaseRotation=off  SenseContactBaseTranslation=off  SenseContactFollowerRotation=off  SenseContactFollowerTranslation=off  ZeroCrossDetectContactStartAndEnd=off
  Contact Force ArmR F2 Block1 : sm_lib/Forces and Torques/Spatial Contact Force  SenseSeparationDistance=off  NormalForceType=SmoothSpringDamper  NormalStiffness=k_gripBox  NormalStiffnessUnits=N/m  NormalDamping=d_gripBox  NormalDampingUnits=N/(m/s)  NormalTransitionRegionWidth=t_gripBox  NormalTransitionRegionWidthUnits=m  FrictionType=SmoothStickSlip  CoefficientOfStaticFriction=mu_s_gripBox  CoefficientOfDynamicFriction=mu_d_gripBox  FrictionalCriticalVelocity=mu_v_gripBox  FrictionalCriticalVelocityUnits=m/s  SenseContactSignal=off  SensePenetrationDepth=off  SenseNormalVelocity=off  SenseTangentialVelocity=off  SensingForceTorqueDirection=BaseOnFollower  SensingForceTorqueResolutionFrame=ContactFrame  SenseNormalForce=off  SenseNormalForceMagnitude=off  SenseNormalTorque=off  SenseFrictionalForce=off  SenseFrictionalForceMagnitude=off  SenseFrictionalTorque=off  SenseTotalForce=off  SenseTotalTorque=off  SenseContactBaseRotation=off  SenseContactBaseTranslation=off  SenseContactFollowerRotation=off  SenseContactFollowerTranslation=off  ZeroCrossDetectContactStartAndEnd=off
  Floor : Subsystem
  Infinite Plane : sm_lib/Curves and Surfaces/Infinite Plane  GraphicType=Rectangle  GraphicPlaneWidth=1  GraphicPlaneWidthUnits=m  GraphicPlaneHeight=1  GraphicPlaneHeightUnits=m  GraphicVisPropType=SimpleVisualProperties  GraphicDiffuseColor=[0.5 0.5 0.5]  GraphicOpacity=0.25  GraphicSpecularColor=[0.5 0.5 0.5 1.0]  GraphicAmbientColor=[0.15 0.15 0.15 1.0]  GraphicEmissiveColor=[0.0 0.0 0.0 1.0]  GraphicShininess=75
  MechanismConfiguration : sm_lib/Utilities/Mechanism Configuration  UniformGravity=Constant  GravityVector=[0 0 -9.80665]  GravityVectorUnits=m/s^2  LinearizationDelta=0.001  JointModeTransitionNonlinearIterations=2
  Simscape Bus : SimscapeBus  HierarchyStrings=F1;F2
  Simscape Bus1 : SimscapeBus  HierarchyStrings=F1;F2
  Solver Configuration : nesl_utility/Solver Configuration  PhysicalDomain=network_engine_domain  SubClassName=solver  LeftPortType=input  RightPortType=generic  Tones=[]  Harmonics=[]  SimulateNoise=off  Profile=off  UseLocalSampling=off  EnableSwitchedLinearOptims=on  FrequencyDomain=off  UseCCode=off  RelTol=0.001  AbsTol=1e-06  MinStep=1e-09  ToWorkspace=off  RevertToSquareIcSolve=off  NumHomotopyIterations=100  PhasorMode=off  PhasorModeNumHarmonics=1  ConsistencySolver=NEWTON_FTOL  IndexReductionMethod=DerivativeReplacement  DoDC=off  ResidualTolerance=1e-09  ConsistencyTolSource=GLOBAL  ConsistencyAbsTol=0.001  ConsistencyRelTol=0.001  ConsistencyTolFactor=0.001  UseLocalSolver=off  LocalSolverChoice=NE_BACKWARD_EULER_ADVANCER  ResolveIndetEquations=on  FunctionEvalNumThread=1  LocalSolverSampleTime=0.001  DoFixedCost=off  MaxNonlinIter=3  MaxModeIter=2  ComputeImpulses=off  ImpulseIterations=2  LinearAlgebra=auto  LinearAlgebraNumThread=0  EquationFormulation=NE_TIME_EF  DelaysMemoryBudget=1024  AutomaticFiltering=on  FilteringTimeConstant=0.001  PartitionStorageMethod=AS_NEEDED  PartitionMemoryBudget=1024  PartitionMethod=ROBUST  MultibodyUseLocalSolver=off  MultibodyLocalSolverChoice=ODE1  MultibodyLocalSolverSampleTime=0.001
  World : sm_lib/Frames and Transforms/World Frame
  Out Bus Element : Outport  PortName=m  Element=trqL
  Out Bus Element1 : Outport  PortName=m  Element=trqR
  wires:
  qR/1 -> Arm R/1(q)
  qL/1 -> Arm L/1(q)
  Arm L/1(trq) -> Out Bus Element/1
  Arm R/1(trq) -> Out Bus Element1/1
  connections:
  6-DOF Joint Block 1/RConn1 -- Block 1/RConn1
  Contact Force ArmL F2 Block1/RConn1 -- Contact Force ArmL F2 Block2/RConn1 -- Block 2/LConn1
  Block 2/LConn2 -- " Contact Force Block to Block"/LConn1 -- Contact Force Block 2 Floor/LConn1
  MechanismConfiguration/RConn1 -- Infinite Plane/LConn1 -- World/RConn1 -- 6-DOF Joint Block 2/LConn1 -- Connection Label1/LConn1 -- Floor/LConn1 -- 6-DOF Joint Block 1/LConn1 -- Solver Configuration/RConn1
  Contact Force ArmR F2 Block1/LConn1 -- Simscape Bus1/LConn2
  Contact Force ArmL F2 Block1/LConn1 -- Simscape Bus/LConn1
  Contact Force ArmR F2 Block1/RConn1 -- " Contact Force Block to Block"/RConn1 -- Block 1/LConn1 -- Contact Force ArmR F1 Block1/RConn1
  Simscape Bus/RConn1 -- Arm L/RConn2
  Contact Force Block 2 Floor/RConn1 -- Contact Force Block 1 Floor/RConn1 -- Infinite Plane/RConn1
  Contact Force Block 1 Floor/LConn1 -- Block 1/LConn2
  Simscape Bus1/RConn1 -- Arm R/RConn1
  Contact Force ArmR F1 Block1/LConn1 -- Simscape Bus1/LConn1
  6-DOF Joint Block 2/RConn1 -- Block 2/RConn1
  Contact Force ArmL F2 Block2/LConn1 -- Simscape Bus/LConn2
  Body/RConn1 -- Arm L/RConn1
  Body/RConn2 -- Arm R/RConn2
  Body/LConn1 -- Connection Label/LConn1
